simulink model "Modulator_DT"  (R2025b)
settings: Solver=FixedStepDiscrete  StartTime=0.0  StopTime=0.5  FixedStep=1/256000  RelTol=1e-3
values from neighbouring files (symbols this model uses):
  a_iir = quantize_coeffs(a_iir_ideal, n_bits)    [bits_quantisation_graph.m]
  b_iir = quantize_coeffs(b_iir_ideal, n_bits)    [bits_quantisation_graph.m]
undefined symbols (not defined in the file or in its folder): dspblkCoreblockFVToolHelper, gcbh
libraries: dspmlti4 x2, dspsrcs4 x1
settings Model: Creator=punee  LastModifiedBy=divijsharma
settings DataIOCC: SaveOutput=off  SignalLogging=off  DSMLogging=off  SaveTime=off  ReturnWorkspaceOutputs=off

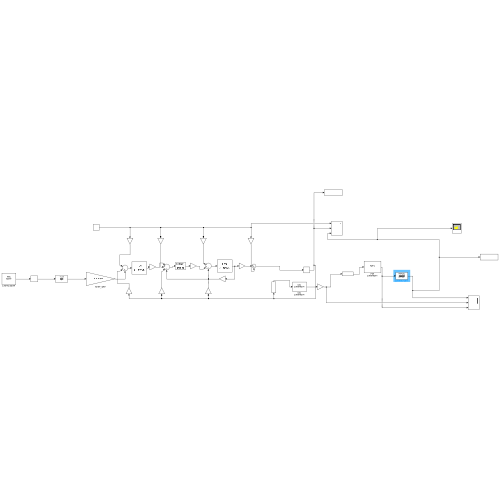
[thumbnail: Simulink's stored preview of the top-level diagram]
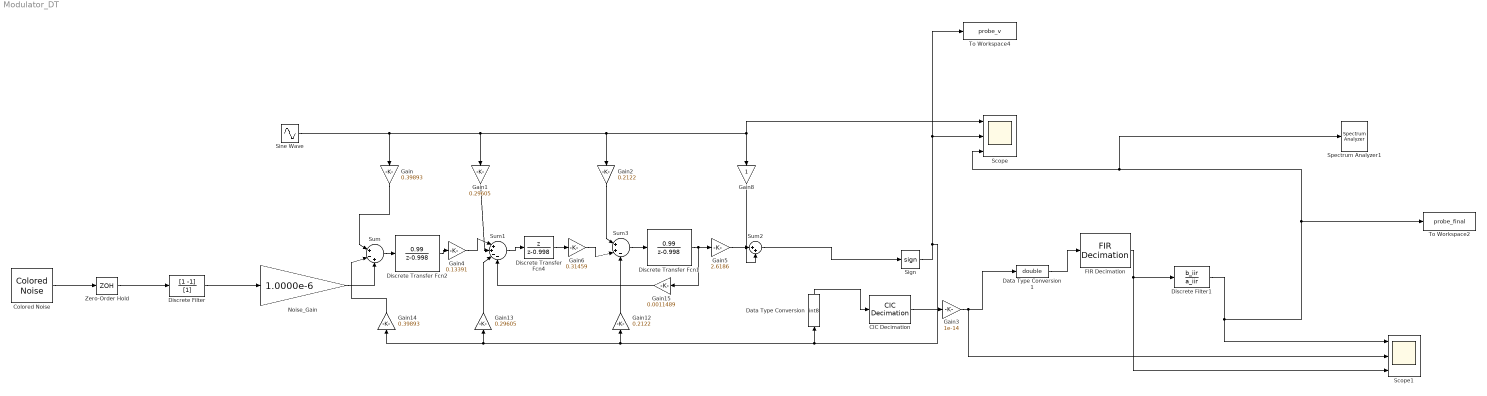
== system Modulator_DT ==
  CIC Decimation : dspmlti4/CIC Decimation  filtFrom=Dialog parameters  filtobj=CICDECIM  ftype=Decimator  R=64  M=1  N=8  filterInternals=Full precision  BPS=[64 64 64 64]  FLPS=0  outputWordLength=32  outputFracLength=0  launchFVT=off  framing=Maintain input frame rate  RateOptions=Allow multirate processing
      settings: LibrarySourceBlock=|
      | dsphdlsupportfiltering/CIC
      | Decimation
  Colored Noise : dspsrcs4/Colored Noise  Color=pink  InverseFrequencyPower=1  BoundedOutput=off  NumChannels=1  OutputDataType=double  SamplesPerFrame=1  SampleTime=1/256000  RandomStream=mt19937ar with seed  Seed=67  SimulateUsing=Interpreted execution
  Data Type Conversion : DataTypeConversion  OutDataTypeStr=int8  RndMeth=Floor
  Data Type Conversion1 : DataTypeConversion  OutDataTypeStr=double  RndMeth=Floor
  Discrete Transfer Fcn1 : DiscreteTransferFcn  LoadFcn=dspblkCoreblockFVToolHelper(gcbh,'load');  Numerator=[0.99]  Denominator=[1 -0.998]
      settings: CopyFcn=dspblkCoreblockFVToolHelper(gcbh,'copy');  DeleteFcn=dspblkCoreblockFVToolHelper(gcbh,'close');  ModelCloseFcn=dspblkCoreblockFVToolHelper(gcbh,'close');  PreSaveFcn=dspblkCoreblockFVToolHelper(gcbh,'presave');  PostSaveFcn=dspblkCoreblockFVToolHelper(gcbh,'postsave');  CloseFcn=dspblkCoreblockFVToolHelper(gcbh,'close');
  Discrete Transfer Fcn2 : DiscreteTransferFcn  LoadFcn=dspblkCoreblockFVToolHelper(gcbh,'load');  Numerator=[0.99]  Denominator=[1 -0.998]
      settings: CopyFcn=dspblkCoreblockFVToolHelper(gcbh,'copy');  DeleteFcn=dspblkCoreblockFVToolHelper(gcbh,'close');  ModelCloseFcn=dspblkCoreblockFVToolHelper(gcbh,'close');  PreSaveFcn=dspblkCoreblockFVToolHelper(gcbh,'presave');  PostSaveFcn=dspblkCoreblockFVToolHelper(gcbh,'postsave');  CloseFcn=dspblkCoreblockFVToolHelper(gcbh,'close');
  Discrete Transfer Fcn4 : DiscreteTransferFcn  LoadFcn=dspblkCoreblockFVToolHelper(gcbh,'load');  Numerator=[1 0]  Denominator=[1 -0.998]
      settings: CopyFcn=dspblkCoreblockFVToolHelper(gcbh,'copy');  DeleteFcn=dspblkCoreblockFVToolHelper(gcbh,'close');  ModelCloseFcn=dspblkCoreblockFVToolHelper(gcbh,'close');  PreSaveFcn=dspblkCoreblockFVToolHelper(gcbh,'presave');  PostSaveFcn=dspblkCoreblockFVToolHelper(gcbh,'postsave');  CloseFcn=dspblkCoreblockFVToolHelper(gcbh,'close');
  Discrete Filter : DiscreteFilter  LoadFcn=dspblkCoreblockFVToolHelper(gcbh,'load');  Numerator=[1 -1]  Denominator=[1]
      settings: CopyFcn=dspblkCoreblockFVToolHelper(gcbh,'copy');  DeleteFcn=dspblkCoreblockFVToolHelper(gcbh,'close');  ModelCloseFcn=dspblkCoreblockFVToolHelper(gcbh,'close');  PreSaveFcn=dspblkCoreblockFVToolHelper(gcbh,'presave');  PostSaveFcn=dspblkCoreblockFVToolHelper(gcbh,'postsave');  CloseFcn=dspblkCoreblockFVToolHelper(gcbh,'close');
  Discrete Filter1 : DiscreteFilter  LoadFcn=dspblkCoreblockFVToolHelper(gcbh,'load');  Numerator=b_iir  Denominator=a_iir
      settings: CopyFcn=dspblkCoreblockFVToolHelper(gcbh,'copy');  DeleteFcn=dspblkCoreblockFVToolHelper(gcbh,'close');  ModelCloseFcn=dspblkCoreblockFVToolHelper(gcbh,'close');  PreSaveFcn=dspblkCoreblockFVToolHelper(gcbh,'presave');  PostSaveFcn=dspblkCoreblockFVToolHelper(gcbh,'postsave');  CloseFcn=dspblkCoreblockFVToolHelper(gcbh,'close');
  FIR Decimation : dspmlti4/FIR Decimation  FilterSource=Dialog parameters  h=b_fir  D=2  filtStruct=Direct form  FilterObject=FDECIM  framing=Allow multirate processing  AllowArbitraryInputLength=off  inputOffset=0  outputBufInitCond=0  roundingMode=Floor  overflowMode=off  firstCoeffDataTypeStr=Inherit: Same word length as input  firstCoeffMin=[]  firstCoeffMax=[]  firstCoeffLastDataTypeStr=Inherit: Same word length as input  outputDataTypeStr=Inherit: Same as accumulator  outputMin=[]  outputMax=[]  outputLastDataTypeStr=Inherit: Same as accumulator
      settings: LibrarySourceBlock=|
      | dsphdlsupportfiltering/FIR
      | Decimation
  Gain : Gain  Gain=0.39893
  Gain1 : Gain  Gain=0.29605
  Gain12 : Gain  Gain=0.2122
  Gain13 : Gain  Gain=0.29605
  Gain14 : Gain  Gain=0.39893
  Gain15 : Gain  Gain=0.0011489
  Gain2 : Gain  Gain=0.2122
  Gain3 : Gain  Gain=1e-14
  Gain4 : Gain  Gain=0.13391
  Gain5 : Gain  Gain=2.6186
  Gain6 : Gain  Gain=0.31459
  Gain8 : Gain
  Noise_Gain : Gain  Gain=1.0000e-6
  Scope : Scope  NumInputPorts=3
      settings: ActiveDisplayYMinimum=-0.75  ActiveDisplayYMaximum=0.75
  Scope1 : Scope  NumInputPorts=3
      settings: ActiveDisplayYMinimum=-2.11919  ActiveDisplayYMaximum=2.07418
  Sign : Signum
  Sine Wave : Sin  Amplitude=0.6  Frequency=2*pi*100  Samples=500  SampleTime=1/256000
  Spectrum Analyzer1 : SpectrumAnalyzer  WindowPosition=[1.000000,1.000000,1280.000000,741.000000,]  ScopeFrameLocation=window  WindowInvariantSamplesPerUpdate=on  Span=2000  StartFrequency=-1000  StopFrequency=1000  YLimits=[-69.0306 5.1962]  SelectedToolstripTab=spectrumAnalyzerToolstrip.measurementsTab
  Sum : Sum  Inputs=|+-+
  Sum1 : Sum  Inputs=|++--
  Sum2 : Sum  Inputs=|++
  Sum3 : Sum  Inputs=|++-
  To Workspace2 : ToWorkspace  VariableName=probe_final  SampleTime=-1
      settings: Save2DSignal=2-D array (concatenate along first dimension)
  To Workspace4 : ToWorkspace  VariableName=probe_v  SampleTime=-1
      settings: Save2DSignal=2-D array (concatenate along first dimension)
  Zero-Order Hold : ZeroOrderHold  SampleTime=1/256000
  wires:
  Gain5/1 -> Sum2/1
  Gain4/1 -> Sum1/1
  Sum3/1 -> Discrete Transfer Fcn1/1
  Gain1/1 -> Sum1/2
  Gain8/1 -> Sum2/2
  Gain13/1 -> Sum1/3
  Gain12/1 -> Sum3/3
  Gain14/1 -> Sum/2
  Discrete Transfer Fcn2/1 -> Gain4/1
  Sum/1 -> Discrete Transfer Fcn2/1
  Sum1/1 -> Discrete Transfer Fcn4/1
  Discrete Transfer Fcn4/1 -> Gain6/1
  Gain15/1 -> Sum1/4
  Gain6/1 -> Sum3/2
  Gain2/1 -> Sum3/1
  Sine Wave/1 -> Gain8/1, Scope/1, Gain2/1, Gain1/1, Gain/1
  CIC Decimation/1 -> Gain3/1
  Colored Noise/1 -> Zero-Order Hold/1
  Sum2/1 -> Sign/1
  Sign/1 -> To Workspace4/1, Scope/2, Data Type Conversion/1, Gain13/1, Gain14/1, Gain12/1
  Data Type Conversion/1 -> CIC Decimation/1
  Gain/1 -> Sum/1
  Zero-Order Hold/1 -> Discrete Filter/1
  Discrete Filter/1 -> Noise_Gain/1
  FIR Decimation/1 -> Scope1/3, Discrete Filter1/1
  Discrete Transfer Fcn1/1 -> Gain15/1, Gain5/1
  Data Type Conversion1/1 -> FIR Decimation/1
  Gain3/1 -> Scope1/2, Data Type Conversion1/1
  Noise_Gain/1 -> Sum/3
  Discrete Filter1/1 -> Scope1/1, Scope/3, Spectrum Analyzer1/1, To Workspace2/1
